simulink model "mdl_with_State_Feedback_integral"  (R2024b)
settings: Solver=VariableStepAuto  StartTime=0.0  StopTime=10.0  RelTol=1e-3
undefined symbols (not defined in the file): input_select, plant_ss, q2_f, Ts
libraries: SignalEditorBlockLib x1
settings Model: Creator=dsagn  LastModifiedBy=dsagn
settings ModelReferenceCC: UpdateModelReferenceTargets=IfOutOfDate
settings SFSimCC: SimGPUStackLimitPerThread=51200
settings RTWCC: GPUStackLimitPerThread=51200  GPUComputeCapability=7.5
settings ConfigComp: CovMetricSettings=de  CovBoundaryAbsTol=1.0e-5

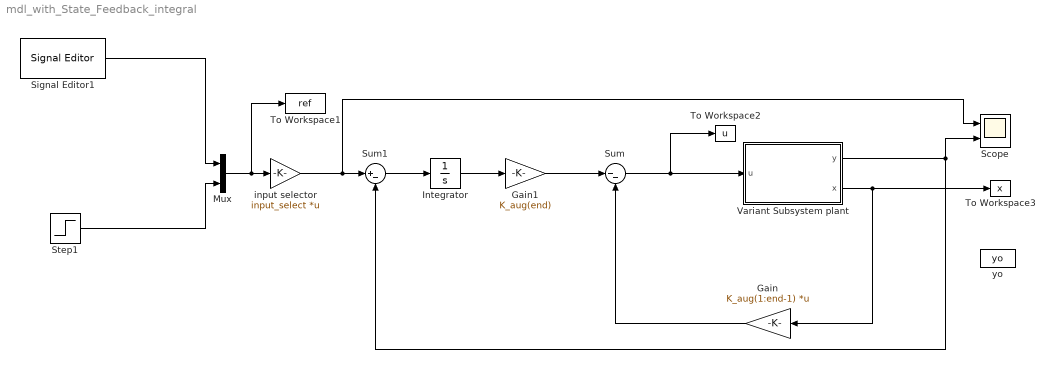
== system mdl_with_State_Feedback_integral ==
  Gain : Gain  Gain=K_aug(1:end-1)  Multiplication=Matrix(K*u) (u vector)
  Gain1 : Gain  Gain=K_aug(end)
  Integrator : Integrator
  Mux : Mux  Inputs=2
  Scope : Scope  NumInputPorts=2
  Signal Editor1 : SignalEditorBlockLib/Signal Editor  FileName=q1_scenario1.mat  ActiveScenario=Scenario  ActiveSignal=Signal 1  IsBus=off  OutputBusObjectStr=Bus: BusObject  SampleTime=Ts  ZeroCross=off  OutputAfterFinalValue=Setting to zero  Unit=inherit  PreserveSignalName=on  ApplySigPropsToAllScenarios=on  ApplySigPropsToAllSignals=off
  Step1 : Step  After=q2_f  SampleTime=Ts
  Sum : Sum  Inputs=|--
  Sum1 : Sum  Inputs=|+-
  To Workspace1 : ToWorkspace  VariableName=ref  SaveFormat=Timeseries  SampleTime=Ts
  To Workspace2 : ToWorkspace  VariableName=u  SaveFormat=Timeseries  SampleTime=-1
  To Workspace3 : ToWorkspace  VariableName=x  SaveFormat=Timeseries  SampleTime=-1
  Variant Subsystem plant : Subsystem  Variant=on
  input selector : Gain  Gain=input_select  Multiplication=Matrix(K*u) (u vector)
  yo : ToWorkspace  VariableName=yo  SaveFormat=Timeseries  SampleTime=-1
  wires:
  input selector/1 -> Sum1/1, Scope/1
  Gain/1 -> Sum/2
  Signal Editor1/1 -> Mux/1
  Sum/1 -> To Workspace2/1, Variant Subsystem plant/1(u)
  Gain1/1 -> Sum/1
  Integrator/1 -> Gain1/1
  Sum1/1 -> Integrator/1
  Variant Subsystem plant/2(x) -> Gain/1, To Workspace3/1
  Variant Subsystem plant/1(y) -> Scope/2, Sum1/2
  Step1/1 -> Mux/2
  Mux/1 -> To Workspace1/1, input selector/1

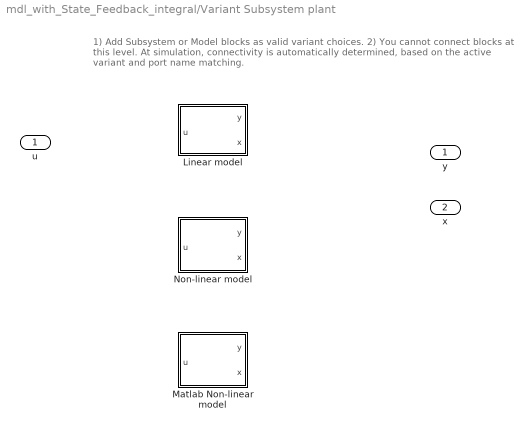
== system mdl_with_State_Feedback_integral/Variant Subsystem plant ==
  note: 1) Add Subsystem or Model blocks as valid variant choices.
      | 2) You cannot connect blocks at this level. At simulation, connectivity is automatically
      | determined, based on the active variant and port name matching.
  u : Inport  SampleTime=Ts
  "Linear model " : Subsystem  VariantControl=model==1
  Matlab Non-linear model : Subsystem  VariantControl=model==3
  Non-linear model : Subsystem  VariantControl=model==2
  y : Outport
  x : Outport  Port=2

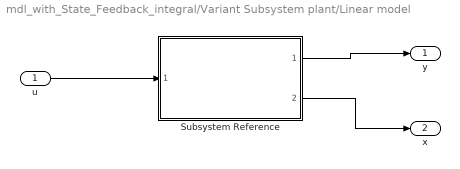
== system mdl_with_State_Feedback_integral/Variant Subsystem plant/Linear model  ==
  u : Inport
  Subsystem Reference : Subsystem  ReferencedSubsystem=pendulum_linear
  y : Outport
  x : Outport  Port=2
  wires:
  u/1 -> Subsystem Reference/1
  Subsystem Reference/1 -> y/1
  Subsystem Reference/2 -> x/1

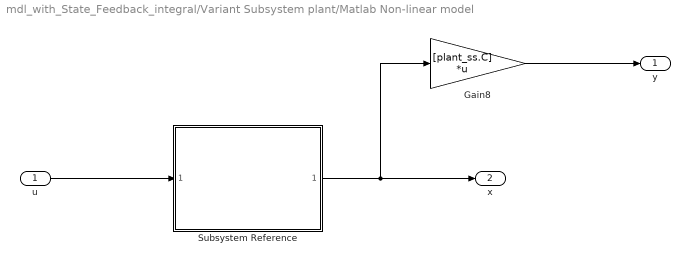
== system mdl_with_State_Feedback_integral/Variant Subsystem plant/Matlab Non-linear model ==
  "u " : Inport  SampleTime=Ts
  Gain8 : Gain  Gain=[plant_ss.C]  Multiplication=Matrix(K*u) (u vector)
  Subsystem Reference : Subsystem  ReferencedSubsystem=pendulum_nonlinear_matlab
  y : Outport  VectorParamsAs1DForOutWhenUnconnected=off
  x : Outport  Port=2
  wires:
  Gain8/1 -> y/1
  Subsystem Reference/1 -> Gain8/1, x/1
  "u "/1 -> Subsystem Reference/1

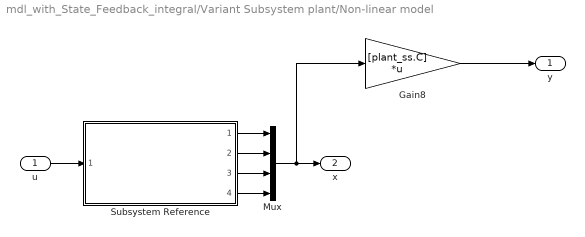
== system mdl_with_State_Feedback_integral/Variant Subsystem plant/Non-linear model ==
  "u " : Inport
  Gain8 : Gain  Gain=[plant_ss.C]  Multiplication=Matrix(K*u) (u vector)
  Mux : Mux
  Subsystem Reference : Subsystem  ReferencedSubsystem=pendulum_nonlinear
  y : Outport  VectorParamsAs1DForOutWhenUnconnected=off
  x : Outport  Port=2
  wires:
  Mux/1 -> Gain8/1, x/1
  Gain8/1 -> y/1
  Subsystem Reference/1 -> Mux/1
  Subsystem Reference/2 -> Mux/2
  Subsystem Reference/3 -> Mux/3
  Subsystem Reference/4 -> Mux/4
  "u "/1 -> Subsystem Reference/1
